simulink model "fimwb_operator_source"  (R2026a)
settings: Solver=FixedStepDiscrete  StopTime=7  FixedStep=1
settings Model: Creator=harry_31916  LastModifiedBy=harry_31916
settings OptimizationCC: BooleanDataType=off

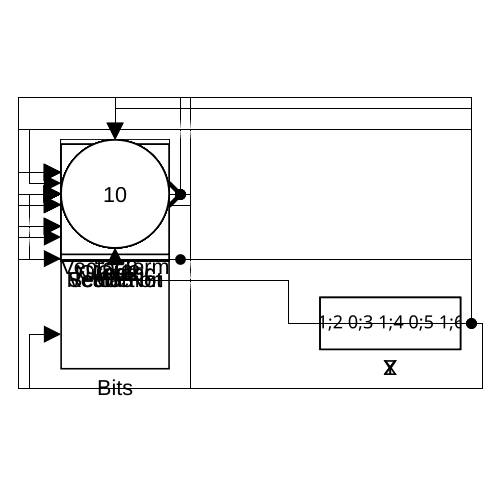
[thumbnail: Simulink's stored preview of the top-level diagram]
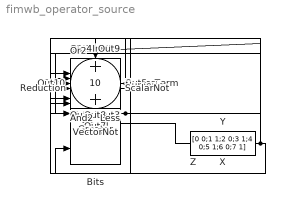
== system fimwb_operator_source ==
  And2 : Logic  AllPortsSameDT=off  OutDataTypeStr=boolean
  Bits : Mux  Inputs=3
  Greater : RelationalOperator  Operator=>
  Less : RelationalOperator  Operator=<
  Minus : Sum  Inputs=--
  Numeric : Logic  Operator=OR  AllPortsSameDT=off
  Or2 : Logic  Operator=OR  AllPortsSameDT=off  OutDataTypeStr=boolean
  Or3 : Logic  Operator=OR  Inputs=3  AllPortsSameDT=off  OutDataTypeStr=boolean
  Plus : Sum
  Reduction : Logic  Inputs=1  AllPortsSameDT=off  OutDataTypeStr=boolean
  ScalarNot : Logic  Operator=NOT  Inputs=1  AllPortsSameDT=off  OutDataTypeStr=boolean
  VectorNot : Logic  Operator=NOT  Inputs=1  AllPortsSameDT=off  OutDataTypeStr=boolean
  VectorTerm : Terminator
  X : FromWorkspace  VariableName=[0 0;1 0;2 0;3 0;4 -2;5 -2;6 2;7 2]  SampleTime=1  Interpolate=off  OutputAfterFinalValue=Holding final value
  XBool : DataTypeConversion  OutDataTypeStr=boolean
  XInt : DataTypeConversion  OutDataTypeStr=int16
  Y : FromWorkspace  VariableName=[0 0;1 0;2 3;3 3;4 0;5 0;6 1;7 1]  SampleTime=1  Interpolate=off  OutputAfterFinalValue=Holding final value
  YBool : DataTypeConversion  OutDataTypeStr=boolean
  YInt : DataTypeConversion  OutDataTypeStr=int16
  Z : FromWorkspace  VariableName=[0 0;1 1;2 0;3 1;4 0;5 1;6 0;7 1]  SampleTime=1  Interpolate=off  OutputAfterFinalValue=Holding final value
  ZBool : DataTypeConversion  OutDataTypeStr=boolean
  ZInt : DataTypeConversion  OutDataTypeStr=int16
  Out1 : Outport
  Out2 : Outport  Port=2
  Out3 : Outport  Port=3
  Out4 : Outport  Port=4
  Out5 : Outport  Port=5
  Out6 : Outport  Port=6
  Out7 : Outport  Port=7
  Out8 : Outport  Port=8
  Out9 : Outport  Port=9
  Out10 : Outport  Port=10
  wires:
  X/1 -> XBool/1, XInt/1, Numeric/1, Plus/1, Minus/1
  Y/1 -> YBool/1, YInt/1, Numeric/2, Plus/2, Minus/2
  Z/1 -> ZBool/1, ZInt/1
  XBool/1 -> Bits/1, And2/1, Or2/1, Or3/1, ScalarNot/1
  YBool/1 -> Bits/2, And2/2, Or2/2, Or3/2
  ZBool/1 -> Bits/3, Or3/3
  Bits/1 -> Reduction/1, VectorNot/1
  VectorNot/1 -> VectorTerm/1
  XInt/1 -> Greater/1, Less/1
  YInt/1 -> Greater/2, Less/2
  And2/1 -> Out1/1
  Or2/1 -> Out2/1
  Or3/1 -> Out3/1
  Numeric/1 -> Out4/1
  Reduction/1 -> Out5/1
  ScalarNot/1 -> Out6/1
  Greater/1 -> Out7/1
  Less/1 -> Out8/1
  Plus/1 -> Out9/1
  Minus/1 -> Out10/1
